simulink model "mppt_boost_switched"  (R2026b)
settings: Solver=ode23t  StopTime=Tstop  MaxStep=Tsw/20  RelTol=1e-4  AbsTol=1e-6
values from neighbouring files (symbols this model uses):
  ctrlMode = 1    [run_switched_validation.m]
  dFixed = opAn.D    [run_switched_validation.m]
  kvec = [K.KpI; K.KiI; K.KpV; K.KiV; Tctrl; bc.dMin; bc.dMax; 40;          round(20e-3/Tctrl); 1.5; Vmp; 20; 250; dFixed; IL0]    [run_switched_validation.m]
  RL = bc.RL    [run_switched_validation.m]
  Tcell = 298.15    [run_switched_validation.m]
  Tctrl = Tsw    [run_switched_validation.m]
  Tsw = 1 / bc.fsw    [run_switched_validation.m]
libraries: fl_lib x11, nesl_utility x7, simulink x1, pvsrc_lib x1
settings Model: Creator=roshh  LastModifiedBy=roshh
settings DataIOCC: SaveOutput=off  SaveTime=off
settings SimscapeCC: SimscapeLogType=all  SimscapeNominalValues="[{\"value\":\"1\",\"unit\":\"A\"},{\"value\":\"1\",\"unit\":\"bar\"},{\"value\":\"1\",\"unit\":\"cm^2\"},{\"value\":\"1\",\"unit\":\"cm^3/s\"},{\"value\":\"1\",\"unit\":\"kJ/kg\"},{\"value\":\"1\",\"unit\":\"kW\"},{\"value\":\"1\",\"unit\":\"l\"},{\"value\":\"1\",\"unit\":\"N\"},{\"value\":\"1\",\"unit\":\"N*m\"},{\"value\":\"1\",\"unit\":\"V\"},{\"value\":\"0.001\",\"unit\":\"Wb\"}]"  SimscapeUseEnergyAccounting=off

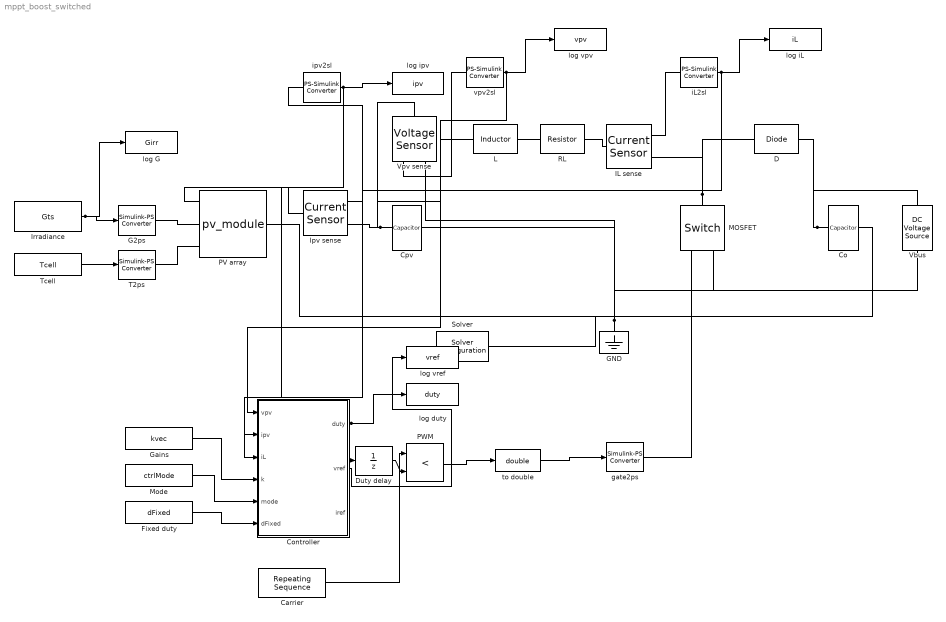
== system mppt_boost_switched ==
  Carrier : simulink/Sources/Repeating Sequence  rep_seq_t=[0 Tsw]  rep_seq_y=[0 1]
  Co : fl_lib/Electrical/Electrical Elements/Capacitor  c=Co F  r=1e-6 Ohm  g=0 1/Ohm  i_specify=off  i_priority=None  i=0 A  i_nominal_specify=off  i_nominal_value=1  i_nominal_unit=A  v_specify=off  v_priority=None  v=0 V  v_nominal_specify=off  v_nominal_value=1  v_nominal_unit=V  vc_specify=off  vc_priority=High  vc=0 V  vc_nominal_specify=off  vc_nominal_value=1  vc_nominal_unit=V
  Controller : MATLAB Function  TreatAsAtomicUnit=on
  Cpv : fl_lib/Electrical/Electrical Elements/Capacitor  c=Cpv F  r=1e-6 Ohm  g=0 1/Ohm  i_specify=off  i_priority=None  i=0 A  i_nominal_specify=off  i_nominal_value=1  i_nominal_unit=A  v_specify=off  v_priority=None  v=0 V  v_nominal_specify=off  v_nominal_value=1  v_nominal_unit=V  vc_specify=off  vc_priority=High  vc=0 V  vc_nominal_specify=off  vc_nominal_value=1  vc_nominal_unit=V
  D : fl_lib/Electrical/Electrical Elements/Diode  Vf=Vf_diode V  Ron=Ron_diode Ohm  Goff=1e-8 1/Ohm  i_specify=off  i_priority=None  i=0 A  i_nominal_specify=off  i_nominal_value=1  i_nominal_unit=A  v_specify=off  v_priority=None  v=0 V  v_nominal_specify=off  v_nominal_value=1  v_nominal_unit=V
  Duty delay : UnitDelay  InitialCondition=dFixed  SampleTime=Tctrl
  Fixed duty : Constant  Value=dFixed
  G2ps : nesl_utility/Simulink-PS Converter  PhysicalDomain=network_engine_domain  SubClassName=ps_input  LeftPortType=input  RightPortType=output  PseudoPeriodic=off  Frequencies=[]  NoiseDistribution=none  NoiseParameters=[]  Unit=W/m^2  AffineConversion=off  FilteringAndDerivatives=provide  SimscapeFilterOrder=1  InputFilterTimeConstant=0.001  UdotUserProvided=0
  GND : fl_lib/Electrical/Electrical Elements/Electrical Reference
  Gains : Constant  Value=kvec
  IL sense : fl_lib/Electrical/Electrical Sensors/Current Sensor
  Ipv sense : fl_lib/Electrical/Electrical Sensors/Current Sensor
  Irradiance : FromWorkspace  VariableName=Gts  OutputAfterFinalValue=Holding final value
  L : fl_lib/Electrical/Electrical Elements/Inductor  l=Lboost H  r=0 Ohm  g=1e-9 1/Ohm  i_specify=off  i_priority=None  i=0 A  i_nominal_specify=off  i_nominal_value=1  i_nominal_unit=A  v_specify=off  v_priority=None  v=0 V  v_nominal_specify=off  v_nominal_value=1  v_nominal_unit=V  i_L_specify=off  i_L_priority=High  i_L=0 A  i_L_nominal_specify=off  i_L_nominal_value=1  i_L_nominal_unit=A
  MOSFET : fl_lib/Electrical/Electrical Elements/Switch  R_closed=Rds_on Ohm  G_open=G_off 1/Ohm  Threshold=0.5  i_specify=off  i_priority=None  i=0 A  i_nominal_specify=off  i_nominal_value=1  i_nominal_unit=A  v_specify=off  v_priority=None  v=0 V  v_nominal_specify=off  v_nominal_value=1  v_nominal_unit=V
  Mode : Constant  Value=ctrlMode
  PV array : pvsrc_lib/pv_module  IphRef=IphRef A  I0Ref=I0Ref A  RsRef=RsRef Ohm  RshRef=RshRef Ohm  aRef=aRef V  alphaIsc=alphaIscPV A/K  EgRef=EgRef  NsMod=NsMod  NpStr=NpStr  i_specify=off  i_priority=None  i=0 A  i_nominal_specify=off  i_nominal_value=1  i_nominal_unit=A  v_specify=off  v_priority=None  v=0 V  v_nominal_specify=off  v_nominal_value=1  v_nominal_unit=V
  PWM : RelationalOperator  Operator=<  OutDataTypeStr=boolean  RndMeth=Simplest  InputSameDT=off
  RL : fl_lib/Electrical/Electrical Elements/Resistor  R=RL Ohm  i_specify=off  i_priority=None  i=0 A  i_nominal_specify=off  i_nominal_value=1  i_nominal_unit=A  v_specify=off  v_priority=None  v=0 V  v_nominal_specify=off  v_nominal_value=1  v_nominal_unit=V
  Solver : nesl_utility/Solver Configuration  PhysicalDomain=network_engine_domain  SubClassName=solver  LeftPortType=input  RightPortType=generic  Tones=[]  Harmonics=[]  SimulateNoise=off  Profile=off  UseLocalSampling=off  EnableSwitchedLinearOptims=on  FrequencyDomain=off  UseCCode=off  RelTol=0.001  AbsTol=0.001  MinStep=1e-09  ToWorkspace=off  RevertToSquareIcSolve=off  NumHomotopyIterations=100  PhasorMode=off  PhasorModeNumHarmonics=1  ConsistencySolver=NEWTON_XTOL_AFTER_FTOL  CanonicalOrdering=CANONICAL  OptimizeIntermediates=OPTIMIZED  MulticoreSolverChoice=BACKWARD_EULER  IndexReductionMethod=DerivativeReplacement  DoDC=off  ResidualTolerance=1e-09  ConsistencyTolSource=GLOBAL  ConsistencyAbsTol=0.001  ConsistencyRelTol=0.001  ConsistencyTolFactor=0.001  UseLocalSolver=off  LocalSolverChoice=NE_BACKWARD_EULER_ADVANCER  ResolveIndetEquations=on  FunctionEvalNumThread=1  LocalSolverSampleTime=0.001  DoFixedCost=off  MaxNonlinIter=3  MaxModeIter=2  ComputeImpulses=off  ImpulseIterations=2  LinearAlgebra=auto  LinearAlgebraNumThread=0  EquationFormulation=NE_TIME_EF  DelaysMemoryBudget=1024  AutomaticFiltering=on  FilteringTimeConstant=0.001  PartitionStorageMethod=AS_NEEDED  PartitionMemoryBudget=1024  PartitionMethod=BALANCED  MultibodyUseLocalSolver=off  MultibodyLocalSolverChoice=ODE1  MultibodyLocalSolverSampleTime=0.001
  T2ps : nesl_utility/Simulink-PS Converter  PhysicalDomain=network_engine_domain  SubClassName=ps_input  LeftPortType=input  RightPortType=output  PseudoPeriodic=off  Frequencies=[]  NoiseDistribution=none  NoiseParameters=[]  Unit=K  AffineConversion=off  FilteringAndDerivatives=provide  SimscapeFilterOrder=1  InputFilterTimeConstant=0.001  UdotUserProvided=0
  Tcell : Constant  Value=Tcell
  Vbus : fl_lib/Electrical/Electrical Sources/DC Voltage Source  v0=Vdc V
  Vpv sense : fl_lib/Electrical/Electrical Sensors/Voltage Sensor
  gate2ps : nesl_utility/Simulink-PS Converter  PhysicalDomain=network_engine_domain  SubClassName=ps_input  LeftPortType=input  RightPortType=output  PseudoPeriodic=off  Frequencies=[]  NoiseDistribution=none  NoiseParameters=[]  Unit=1  AffineConversion=off  FilteringAndDerivatives=provide  SimscapeFilterOrder=1  InputFilterTimeConstant=0.001  UdotUserProvided=0
  iL2sl : nesl_utility/PS-Simulink Converter  PhysicalDomain=network_engine_domain  SubClassName=ps_output  LeftPortType=input  RightPortType=output  PseudoPeriodic=off  Frequencies=[]  VectorFormat=inherit  Unit=A  AffineConversion=off
  ipv2sl : nesl_utility/PS-Simulink Converter  PhysicalDomain=network_engine_domain  SubClassName=ps_output  LeftPortType=input  RightPortType=output  PseudoPeriodic=off  Frequencies=[]  VectorFormat=inherit  Unit=A  AffineConversion=off
  log G : ToWorkspace  VariableName=Girr  SaveFormat=Structure With Time  SampleTime=-1
  log duty : ToWorkspace  VariableName=duty  SaveFormat=Structure With Time  SampleTime=-1
  log iL : ToWorkspace  VariableName=iL  SaveFormat=Structure With Time  SampleTime=-1
  log ipv : ToWorkspace  VariableName=ipv  SaveFormat=Structure With Time  SampleTime=-1
  log vpv : ToWorkspace  VariableName=vpv  SaveFormat=Structure With Time  SampleTime=-1
  log vref : ToWorkspace  VariableName=vref  SaveFormat=Structure With Time  SampleTime=-1
  to double : DataTypeConversion  OutDataTypeStr=double  SaturateOnIntegerOverflow=off  RndMeth=Floor
  vpv2sl : nesl_utility/PS-Simulink Converter  PhysicalDomain=network_engine_domain  SubClassName=ps_output  LeftPortType=input  RightPortType=output  PseudoPeriodic=off  Frequencies=[]  VectorFormat=inherit  Unit=V  AffineConversion=off
  wires:
  Irradiance/1 -> G2ps/1, log G/1
  Tcell/1 -> T2ps/1
  vpv2sl/1 -> Controller/1(vpv), log vpv/1
  ipv2sl/1 -> Controller/2(ipv), log ipv/1
  iL2sl/1 -> Controller/3(iL), log iL/1
  Gains/1 -> Controller/4(k)
  Mode/1 -> Controller/5(mode)
  Fixed duty/1 -> Controller/6(dFixed)
  Carrier/1 -> PWM/1
  Controller/1(duty) -> Duty delay/1, log duty/1
  Duty delay/1 -> PWM/2
  PWM/1 -> to double/1
  to double/1 -> gate2ps/1
  Controller/2(vref) -> log vref/1
  connections:
  PV array/LConn1 -- Ipv sense/LConn1
  Ipv sense/RConn2 -- Vpv sense/LConn1 -- Cpv/LConn1 -- L/LConn1
  PV array/RConn1 -- Cpv/RConn1 -- Vpv sense/RConn2 -- MOSFET/RConn2 -- Co/RConn1 -- Vbus/RConn1 -- GND/LConn1 -- Solver/RConn1
  L/RConn1 -- RL/LConn1
  RL/RConn1 -- IL sense/LConn1
  MOSFET/LConn1 -- IL sense/RConn2 -- D/LConn1
  Co/LConn1 -- D/RConn1 -- Vbus/LConn1
  G2ps/RConn1 -- PV array/LConn2
  T2ps/RConn1 -- PV array/LConn3
  Ipv sense/RConn1 -- ipv2sl/LConn1
  Vpv sense/RConn1 -- vpv2sl/LConn1
  IL sense/RConn1 -- iL2sl/LConn1
  gate2ps/RConn1 -- MOSFET/RConn1

== matlab function mppt_boost_switched/Controller ==
  settings: updateMethod=DISCRETE  sampleTime=Tctrl
  data: vpv input; duty output; ipv input; iL input; k input; mode input; dFixed input; vref output; iref output
function [duty, vref, iref] = controller(vpv, ipv, iL, k, mode, dFixed)
persistent xi xv Vref cnt Pprev dirn ready
KpI = k(1); KiI = k(2); KpV = k(3); KiV = k(4); Ts = k(5);
dMin = k(6); dMax = k(7); ILmax = k(8); nM = k(9); step = k(10);
V0 = k(11); Vlo = k(12); Vhi = k(13);
if isempty(ready)
    ready = true; xi = k(14); xv = k(15); Vref = V0; cnt = 0; Pprev = -1; dirn = 1;
end
if mode > 0.5
    cnt = cnt + 1;
    if cnt >= nM
        cnt = 0;
        Pnow = vpv * ipv;
        if Pprev >= 0 && Pnow < Pprev
            dirn = -dirn;
        end
        Vref = Vref + dirn * step;
        Pprev = Pnow;
    end
end
if Vref < Vlo, Vref = Vlo; end
if Vref > Vhi, Vref = Vhi; end
ev = vpv - Vref;
rawI = KpV*ev + xv;
iref = min(max(rawI, 0), ILmax);
xv = xv + Ts*(KiV*ev + (KiV/KpV)*(iref - rawI));
ei = iref - iL;
rawD = KpI*ei + xi;
duty = min(max(rawD, dMin), dMax);
xi = xi + Ts*(KiI*ei + (KiI/KpI)*(duty - rawD));
if mode < -0.5
    duty = dFixed;
end
vref = Vref;
